simulink model "Q5_4_4_A"  (R2023b)
settings: Solver=ode4  StartTime=0.0  StopTime=10  FixedStep=1e-4  RelTol=1e-3
settings Model: Creator=Arshia  LastModifiedBy=Arshia

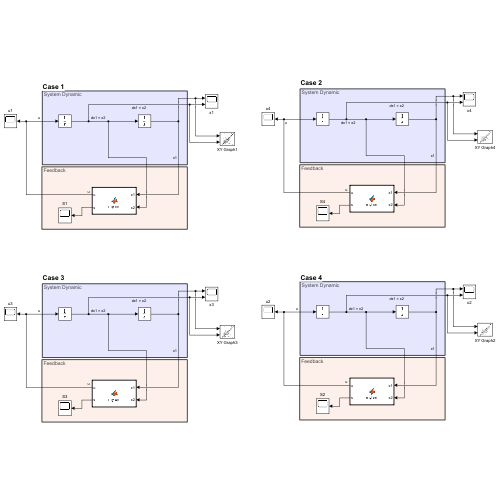
[thumbnail: Simulink's stored preview of the top-level diagram]
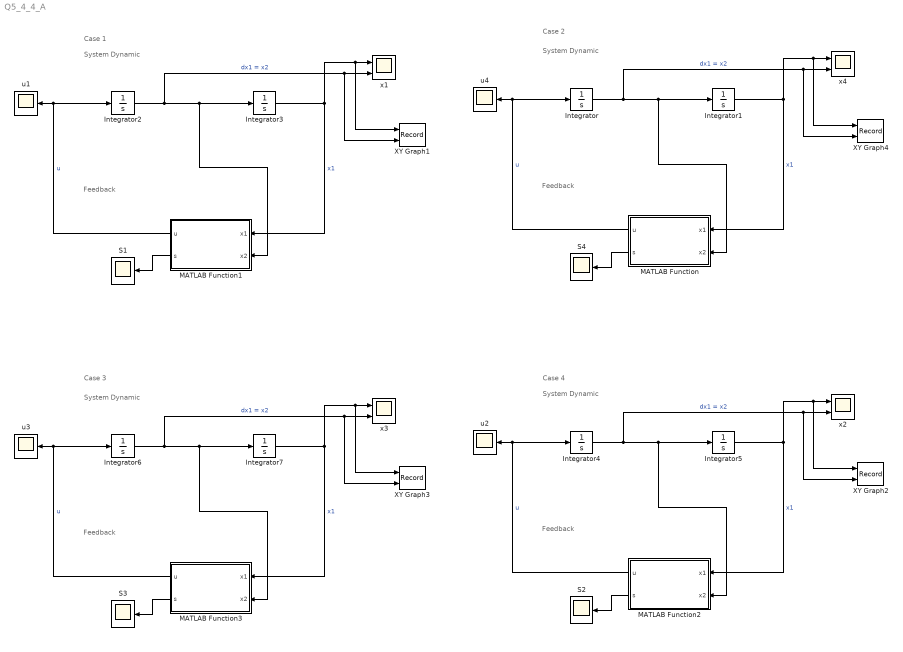
== system Q5_4_4_A ==
  note: Case 1
  note: Feedback
  note: System Dynamic
  note: System Dynamic
  note: Feedback
  note: Feedback
  note: System Dynamic
  note: System Dynamic
  note: Feedback
  note: Case 2
  note: Case 3
  note: Case 4
  Integrator{,3..4,6} (4 alike) : Integrator  InitialCondition=-2
  Integrator1 : Integrator  InitialCondition=2
  Integrator2 : Integrator  InitialCondition=2
  Integrator5 : Integrator  InitialCondition=-4
  Integrator7 : Integrator  InitialCondition=4
  MATLAB Function : MATLAB Function  TreatAsAtomicUnit=on
  MATLAB Function1 : MATLAB Function  TreatAsAtomicUnit=on
  MATLAB Function2 : MATLAB Function  TreatAsAtomicUnit=on
  MATLAB Function3 : MATLAB Function  TreatAsAtomicUnit=on
  S{1..4} (4 alike) : Scope
  XY Graph1 : Record  FileSettingsInternal="{\"entries\":[{\"content\":{\"excelSettings\":{\"content\":{},\"type\":\"Streamout.ExcelSettings\"}},\"type\":\"Streamout.FileSettingStorage\",\"uuid\":\"\"}],\"packageUris\":[\"http:\\/\\/schema.mathworks.com\\/mf0\\/streamout_blocks\\/R2020a\"],\"version\":\"1.0\"}"  Layout=[1 1]  SignalsInternal="{\"entries\":[{\"content\":{\"signals\":[{\"content\":{\"blockPath\":[],\"dimensions\":[1],\"domain\":\"\",\"lineColor\":\"#a2142f\",\"plots\":[ 1 ],\"port\":1,\"signalID\":1,\"signalName\":\"x1\"},\"type\":\"RecordBlkView.Signal\",\"uuid\":\"\"},{\"content\":{\"blockPath\":[],\"dimensions\":[1],\"domain\":\"\",\"lineColor\":\"#139fff\",\"plots\":[ 1 ],\"port\":2,\"signalID\":2,\"signalName\":\"dx1 = x2\"},\"type\":\"RecordBlkView.Signal\",\"uuid\":\"\"}]},\"type\":\"RecordBlkView.InputSignals\",\"uuid\":\"\"}],\"packageUris\":[\"http:\\/\\/schema.mathworks.com\\/mf0\\/streamout_blocks\\/R2020a\"],\"version\":\"1.0\"}"  VisualizationBindings="{\"xyplotplugin\":{\"info\":[{\"series\":[{\"bindingParametersList\":[{\"parameter\":\"X-Axis\",\"signalID\":1,\"signalName\":\"x1\"},{\"parameter\":\"Y-Axis\",\"signalID\":2,\"signalName\":\"dx1 = x2\"}],\"seriesID\":0}],\"subplotID\":1}]}}"  CompatibilityTag=XY
  XY Graph2 : Record  FileSettingsInternal="{\"entries\":[{\"content\":{\"excelSettings\":{\"content\":{},\"type\":\"Streamout.ExcelSettings\"}},\"type\":\"Streamout.FileSettingStorage\",\"uuid\":\"\"}],\"packageUris\":[\"http:\\/\\/schema.mathworks.com\\/mf0\\/streamout_blocks\\/R2020a\"],\"version\":\"1.0\"}"  Layout=[1 1]  SignalsInternal="{\"entries\":[{\"content\":{\"signals\":[{\"content\":{\"blockPath\":[],\"dimensions\":[1],\"domain\":\"\",\"lineColor\":\"#a2142f\",\"plots\":[ 1 ],\"port\":1,\"signalID\":1,\"signalName\":\"x1\"},\"type\":\"RecordBlkView.Signal\",\"uuid\":\"\"},{\"content\":{\"blockPath\":[],\"dimensions\":[1],\"domain\":\"\",\"lineColor\":\"#139fff\",\"plots\":[ 1 ],\"port\":2,\"signalID\":2,\"signalName\":\"dx1 = x2\"},\"type\":\"RecordBlkView.Signal\",\"uuid\":\"\"}]},\"type\":\"RecordBlkView.InputSignals\",\"uuid\":\"\"}],\"packageUris\":[\"http:\\/\\/schema.mathworks.com\\/mf0\\/streamout_blocks\\/R2020a\"],\"version\":\"1.0\"}"  VisualizationBindings="{\"xyplotplugin\":{\"info\":[{\"series\":[{\"bindingParametersList\":[{\"parameter\":\"X-Axis\",\"signalID\":1,\"signalName\":\"x1\"},{\"parameter\":\"Y-Axis\",\"signalID\":2,\"signalName\":\"dx1 = x2\"}],\"seriesID\":0}],\"subplotID\":1}]}}"  CompatibilityTag=XY
  XY Graph3 : Record  FileSettingsInternal="{\"entries\":[{\"content\":{\"excelSettings\":{\"content\":{},\"type\":\"Streamout.ExcelSettings\"}},\"type\":\"Streamout.FileSettingStorage\",\"uuid\":\"\"}],\"packageUris\":[\"http:\\/\\/schema.mathworks.com\\/mf0\\/streamout_blocks\\/R2020a\"],\"version\":\"1.0\"}"  Layout=[1 1]  SignalsInternal="{\"entries\":[{\"content\":{\"signals\":[{\"content\":{\"blockPath\":[],\"dimensions\":[1],\"domain\":\"\",\"lineColor\":\"#a2142f\",\"plots\":[ 1 ],\"port\":1,\"signalID\":1,\"signalName\":\"x1\"},\"type\":\"RecordBlkView.Signal\",\"uuid\":\"\"},{\"content\":{\"blockPath\":[],\"dimensions\":[1],\"domain\":\"\",\"lineColor\":\"#139fff\",\"plots\":[ 1 ],\"port\":2,\"signalID\":2,\"signalName\":\"dx1 = x2\"},\"type\":\"RecordBlkView.Signal\",\"uuid\":\"\"}]},\"type\":\"RecordBlkView.InputSignals\",\"uuid\":\"\"}],\"packageUris\":[\"http:\\/\\/schema.mathworks.com\\/mf0\\/streamout_blocks\\/R2020a\"],\"version\":\"1.0\"}"  VisualizationBindings="{\"xyplotplugin\":{\"info\":[{\"series\":[{\"bindingParametersList\":[{\"parameter\":\"X-Axis\",\"signalID\":1,\"signalName\":\"x1\"},{\"parameter\":\"Y-Axis\",\"signalID\":2,\"signalName\":\"dx1 = x2\"}],\"seriesID\":0}],\"subplotID\":1}]}}"  CompatibilityTag=XY
  XY Graph4 : Record  FileSettingsInternal="{\"entries\":[{\"content\":{\"excelSettings\":{\"content\":{},\"type\":\"Streamout.ExcelSettings\"}},\"type\":\"Streamout.FileSettingStorage\",\"uuid\":\"\"}],\"packageUris\":[\"http:\\/\\/schema.mathworks.com\\/mf0\\/streamout_blocks\\/R2020a\"],\"version\":\"1.0\"}"  Layout=[1 1]  SignalsInternal="{\"entries\":[{\"content\":{\"signals\":[{\"content\":{\"blockPath\":[],\"dimensions\":[1],\"domain\":\"\",\"lineColor\":\"#64d413\",\"port\":1,\"signalID\":1,\"signalName\":\"x1\"},\"type\":\"RecordBlkView.Signal\",\"uuid\":\"\"},{\"content\":{\"blockPath\":[],\"dimensions\":[1],\"domain\":\"\",\"lineColor\":\"#ff13a6\",\"port\":2,\"signalID\":2,\"signalName\":\"dx1 = x2\"},\"type\":\"RecordBlkView.Signal\",\"uuid\":\"\"}]},\"type\":\"RecordBlkView.InputSignals\",\"uuid\":\"\"}],\"packageUris\":[\"http:\\/\\/schema.mathworks.com\\/mf0\\/streamout_blocks\\/R2020a\"],\"version\":\"1.0\"}"  VisualizationBindings="{\"xyplotplugin\":{\"info\":[{\"series\":[],\"subplotID\":1}]}}"  CompatibilityTag=XY
  u{1..4} (4 alike) : Scope
  x{1..4} (4 alike) : Scope  NumInputPorts=2
  wires:
  MATLAB Function/1(u) -> Integrator/1, u4/1  "u"
  Integrator/1 -> Integrator1/1, MATLAB Function/2(x2), XY Graph4/2, x4/2  "dx1 = x2"
  Integrator1/1 -> MATLAB Function/1(x1), XY Graph4/1, x4/1  "x1"
  MATLAB Function/2(s) -> S4/1
  MATLAB Function1/2(s) -> S1/1
  Integrator2/1 -> Integrator3/1, MATLAB Function1/2(x2), XY Graph1/2, x1/2  "dx1 = x2"
  MATLAB Function1/1(u) -> Integrator2/1, u1/1  "u"
  Integrator3/1 -> MATLAB Function1/1(x1), XY Graph1/1, x1/1  "x1"
  Integrator7/1 -> MATLAB Function3/1(x1), XY Graph3/1, x3/1  "x1"
  MATLAB Function3/2(s) -> S3/1
  Integrator6/1 -> Integrator7/1, MATLAB Function3/2(x2), XY Graph3/2, x3/2  "dx1 = x2"
  MATLAB Function2/2(s) -> S2/1
  MATLAB Function3/1(u) -> Integrator6/1, u3/1  "u"
  Integrator4/1 -> Integrator5/1, MATLAB Function2/2(x2), XY Graph2/2, x2/2  "dx1 = x2"
  MATLAB Function2/1(u) -> Integrator4/1, u2/1  "u"
  Integrator5/1 -> MATLAB Function2/1(x1), XY Graph2/1, x2/1  "x1"

== matlab function Q5_4_4_A/MATLAB Function1 ==
  data: u output; x1 input; x2 input; s output
function [u, s] = myfcn(x1, x2)
s = x1 + 0.5 * x2 * abs(x2);
u = 0;
eps1 = 1e-3;
eps2 = 1e-4;  
if abs(x1) < eps2 && abs(x2) < eps2
    u = 0;  
else
    if s > eps1
        u = -1;
    elseif s < -eps1
        u = +1;
    elseif abs(s) <= eps1
        if x2 > eps2
            u = -1;
        elseif x2 < -eps2
            u = +1;
        else
            u = 0;
        end
    end
end
end

== matlab function Q5_4_4_A/MATLAB Function ==
  data: u output; x1 input; x2 input; s output
function [u, s] = myfcn(x1, x2)
s = x1 + 0.5 * x2 * abs(x2);
u = 0;
eps1 = 1e-3;
eps2 = 1e-4;  
if abs(x1) < eps2 && abs(x2) < eps2
    u = 0;  
else
    if s > eps1
        u = -1;
    elseif s < -eps1
        u = +1;
    elseif abs(s) <= eps1
        if x2 > eps2
            u = -1;
        elseif x2 < -eps2
            u = +1;
        else
            u = 0;
        end
    end
end
end

== matlab function Q5_4_4_A/MATLAB Function2 ==
  data: u output; x1 input; x2 input; s output
function [u, s] = myfcn(x1, x2)
s = x1 + 0.5 * x2 * abs(x2);
u = 0;
eps1 = 1e-3;
eps2 = 1e-4;  
if abs(x1) < eps2 && abs(x2) < eps2
    u = 0;  
else
    if s > eps1
        u = -1;
    elseif s < -eps1
        u = +1;
    elseif abs(s) <= eps1
        if x2 > eps2
            u = -1;
        elseif x2 < -eps2
            u = +1;
        else
            u = 0;
        end
    end
end
end

== matlab function Q5_4_4_A/MATLAB Function3 ==
  data: u output; x1 input; x2 input; s output
function [u, s] = myfcn(x1, x2)
s = x1 + 0.5 * x2 * abs(x2);
u = 0;
eps1 = 1e-3;
eps2 = 1e-4;  
if abs(x1) < eps2 && abs(x2) < eps2
    u = 0;  
else
    if s > eps1
        u = -1;
    elseif s < -eps1
        u = +1;
    elseif abs(s) <= eps1
        if x2 > eps2
            u = -1;
        elseif x2 < -eps2
            u = +1;
        else
            u = 0;
        end
    end
end
end
